simulink library "bq76952Decode_lib"  (R2025b)
settings: Solver=VariableStepAuto  StartTime=0.0  StopTime=10.0  RelTol=1e-3
libraries: $bdroot x6, simulink x2
settings Model: Creator=SC-Br  LastModifiedBy=SC-Br

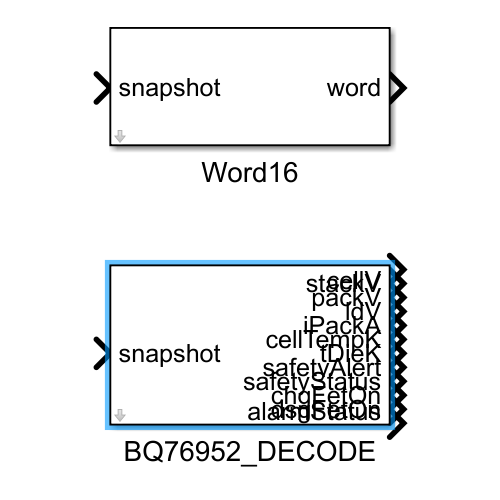
[thumbnail: Simulink's stored preview of the top-level diagram]
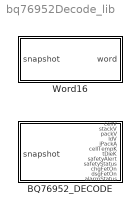
== system bq76952Decode_lib ==
  BQ76952_DECODE : Subsystem  mask{DAConfig=6, cellMap=[1 2 3 16], thermPins=[4 6 7 8]}
      mask prompts: DAConfig "DA_CONFIG (must match EVM)"; cellMap "Used cell channels"; thermPins "Thermistor pins (cell order)"
  Word16 : Subsystem  mask{regs=hex2dec('14') + 2*(0:15), isSigned=1}
      mask prompts: regs "Register addresses"; isSigned "Signed (1/0)"

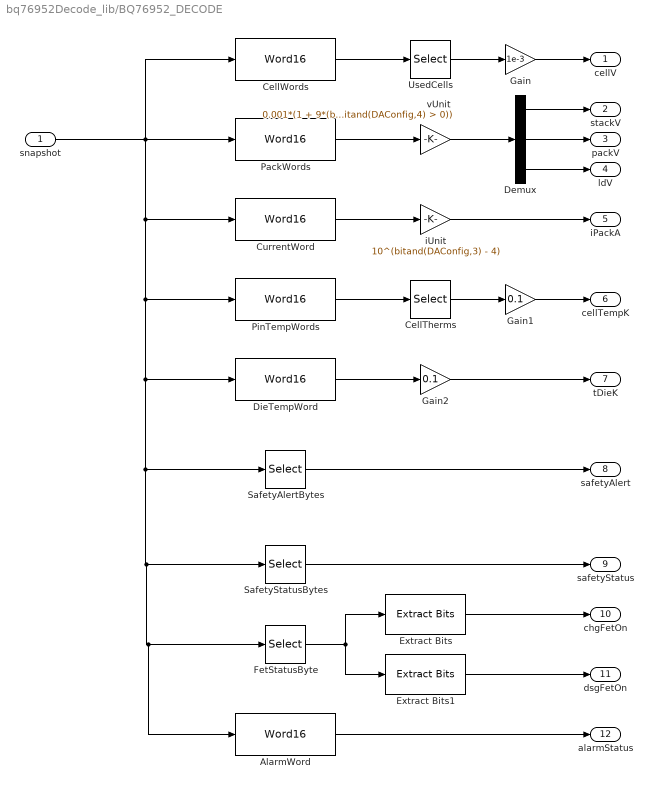
== system bq76952Decode_lib/BQ76952_DECODE ==
  snapshot : Inport
  AlarmWord : $bdroot/Word16  regs=hex2dec('62')  isSigned=0
  CellTherms : Selector  InputPortWidth=9  IndexOptions=Index vector (dialog)  Indices=thermPins  OutputSizes=1
  CellWords : $bdroot/Word16  regs=hex2dec('14') + 2*(0:15)  isSigned=1
  CurrentWord : $bdroot/Word16  regs=hex2dec('3A')  isSigned=1
  Demux : Demux  Outputs=3
  DieTempWord : $bdroot/Word16  regs=hex2dec('68')  isSigned=1
  Extract Bits : simulink/Logic and Bit Operations/Extract Bits  bitsToExtract=Range of bits  numBits=8  bitIdxRange=[0 0]  outScalingMode=Treat bit field as an integer
  Extract Bits1 : simulink/Logic and Bit Operations/Extract Bits  bitsToExtract=Range of bits  numBits=8  bitIdxRange=[2 2]  outScalingMode=Treat bit field as an integer
  FetStatusByte : Selector  InputPortWidth=144  IndexOptions=Index vector (dialog)  Indices=144  OutputSizes=1
  Gain : Gain  Gain=1e-3
  Gain1 : Gain  Gain=0.1
  Gain2 : Gain  Gain=0.1
  PackWords : $bdroot/Word16  regs=hex2dec({'34';'36';'38'})  isSigned=1
  PinTempWords : $bdroot/Word16  regs=hex2dec('6A') + 2*(0:8)  isSigned=1
  SafetyAlertBytes : Selector  InputPortWidth=144  IndexOptions=Index vector (dialog)  Indices=[19 21 23]  OutputSizes=1
  SafetyStatusBytes : Selector  InputPortWidth=144  IndexOptions=Index vector (dialog)  Indices=[19 21 23]  OutputSizes=1
  UsedCells : Selector  InputPortWidth=16  IndexOptions=Index vector (dialog)  Indices=cellMap  OutputSizes=1
  iUnit : Gain  Gain=10^(bitand(DAConfig,3) - 4)
  vUnit : Gain  Gain=0.001*(1 + 9*(bitand(DAConfig,4) > 0))
  cellV : Outport
  stackV : Outport  Port=2
  packV : Outport  Port=3
  ldV : Outport  Port=4
  iPackA : Outport  Port=5
  cellTempK : Outport  Port=6
  tDieK : Outport  Port=7
  safetyAlert : Outport  Port=8
  safetyStatus : Outport  Port=9
  chgFetOn : Outport  Port=10
  dsgFetOn : Outport  Port=11
  alarmStatus : Outport  Port=12
  wires:
  UsedCells/1 -> Gain/1
  vUnit/1 -> Demux/1
  Gain/1 -> cellV/1
  Demux/1 -> stackV/1
  Demux/2 -> packV/1
  Demux/3 -> ldV/1
  iUnit/1 -> iPackA/1
  CurrentWord/1 -> iUnit/1
  PackWords/1 -> vUnit/1
  CellWords/1 -> UsedCells/1
  PinTempWords/1 -> CellTherms/1
  DieTempWord/1 -> Gain2/1
  Gain1/1 -> cellTempK/1
  Gain2/1 -> tDieK/1
  CellTherms/1 -> Gain1/1
  SafetyAlertBytes/1 -> safetyAlert/1
  snapshot/1 -> AlarmWord/1, FetStatusByte/1, SafetyStatusBytes/1, SafetyAlertBytes/1, DieTempWord/1, PinTempWords/1, CurrentWord/1, PackWords/1, CellWords/1
  SafetyStatusBytes/1 -> safetyStatus/1
  AlarmWord/1 -> alarmStatus/1
  FetStatusByte/1 -> Extract Bits1/1, Extract Bits/1
  Extract Bits/1 -> chgFetOn/1
  Extract Bits1/1 -> dsgFetOn/1

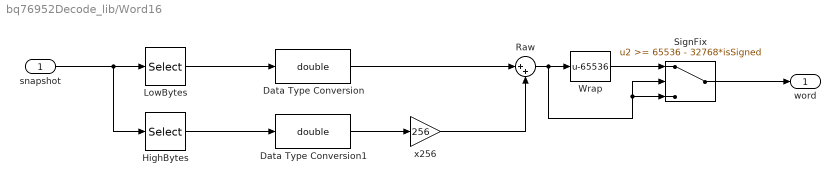
== system bq76952Decode_lib/Word16 ==
  snapshot : Inport
  Data Type Conversion : DataTypeConversion  OutDataTypeStr=double  SaturateOnIntegerOverflow=off  RndMeth=Floor
  Data Type Conversion1 : DataTypeConversion  OutDataTypeStr=double  SaturateOnIntegerOverflow=off  RndMeth=Floor
  HighBytes : Selector  InputPortWidth=144  IndexOptions=Index vector (dialog)  Indices=18 + regs  OutputSizes=1
  LowBytes : Selector  InputPortWidth=144  IndexOptions=Index vector (dialog)  Indices=17 + regs  OutputSizes=1
  Raw : Sum  Inputs=|++
  SignFix : Switch  Threshold=65536 - 32768*isSigned  SaturateOnIntegerOverflow=off  InputSameDT=off
  Wrap : Bias  Bias=-65536  SaturateOnIntegerOverflow=off
  x256 : Gain  Gain=256
  word : Outport
  wires:
  HighBytes/1 -> Data Type Conversion1/1
  LowBytes/1 -> Data Type Conversion/1
  SignFix/1 -> word/1
  Wrap/1 -> SignFix/1
  Raw/1 -> Wrap/1, SignFix/2, SignFix/3
  x256/1 -> Raw/2
  Data Type Conversion1/1 -> x256/1
  Data Type Conversion/1 -> Raw/1
  snapshot/1 -> LowBytes/1, HighBytes/1
